simulink model "ABS_VehicleSpeed_Model"  (R2025a)
settings: Solver=VariableStepAuto  StartTime=0.0  StopTime=10.0  RelTol=1e-3
settings Model: Creator=nikul  LastModifiedBy=nikul

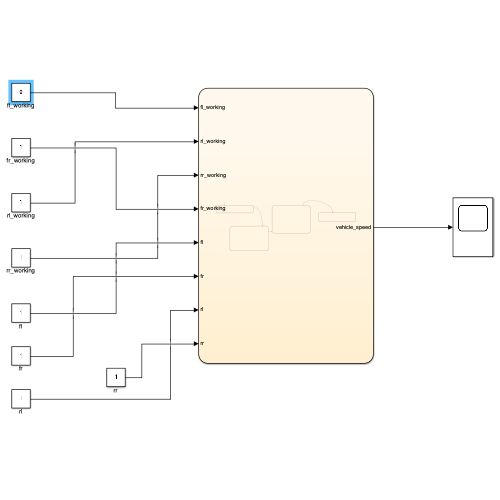
[thumbnail: Simulink's stored preview of the top-level diagram]
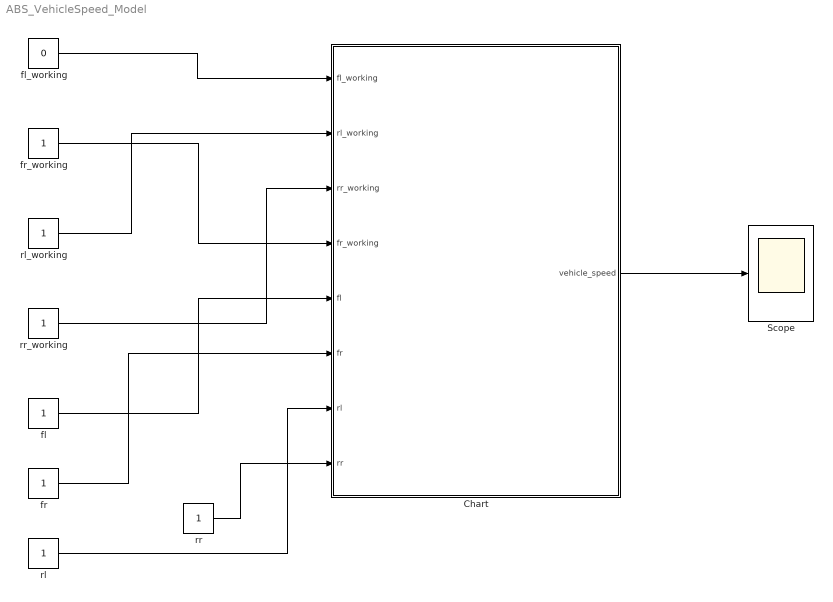
== system ABS_VehicleSpeed_Model ==
  Chart : Stateflow chart  TreatAsAtomicUnit=on
  Scope : Scope
  fl : Constant  OutDataTypeStr=double
  fl_working : Constant  Value=0  OutDataTypeStr=boolean
  fr : Constant  OutDataTypeStr=double
  fr_working : Constant  OutDataTypeStr=boolean
  rl : Constant  OutDataTypeStr=double
  rl_working : Constant  OutDataTypeStr=boolean
  rr : Constant  OutDataTypeStr=double
  rr_working : Constant  OutDataTypeStr=boolean
  wires:
  fl_working/1 -> Chart/1(fl_working)
  fr_working/1 -> Chart/4(fr_working)
  rl_working/1 -> Chart/2(rl_working)
  rr_working/1 -> Chart/3(rr_working)
  fl/1 -> Chart/5(fl)
  fr/1 -> Chart/6(fr)
  rl/1 -> Chart/7(rl)
  rr/1 -> Chart/8(rr)
  Chart/1(vehicle_speed) -> Scope/1

== stateflow chart ABS_VehicleSpeed_Model/Chart ==
  state AllSensorsWorking
    fl_working && fr_working && rl_working && rr_working
    vehicle_speed = (fl + fr + rl + rr) / 4;
  state TwoSensorsDown
    (fl_working + fr_working + rl_working + rr_working) == 2
    if fl_working && fr_working
    vehicle_speed = (fl + fr)/2;
    elseif fl_working && rl_working
    vehicle_speed = (fl + rl)/2;
    elseif fl_working && rr_working
    vehicle_speed = (fl + rr)/2;
    elseif fr_working && rl_working
    vehicle_speed = (fr + rl)/2;
    elseif fr_working && rr_working
    vehicle_speed = (fr + rr)/2;
    elseif rl_working && rr_working
    vehicle_speed = (rl + rr)/2;
    end
  state ThreeOrMoreDown
    (fl_working + fr_working + rl_working + rr_working) <= 1
    vehicle_speed = 0;
  state OneSensorDown
    (~fl_working && fr_working && rl_working && rr_working)
    (~fr_working && fl_working && rl_working && rr_working)
    (~rl_working && fl_working && fr_working && rr_working)
    (~rr_working && fl_working && fr_working && rl_working)
    if ~fl_working
    vehicle_speed = (fr + rl + rr)/3;
    elseif ~fr_working
    vehicle_speed = (fl + rl + rr)/3;
    elseif ~rl_working
    vehicle_speed = (fl + fr + rr)/3;
    elseif ~rr_working
    vehicle_speed = (fl + fr + rl)/3;
    end
  TwoSensorsDown -> ThreeOrMoreDown
  (default) -> AllSensorsWorking
  AllSensorsWorking -> OneSensorDown
  OneSensorDown -> TwoSensorsDown
  data: fl_working input boolean; rl_working input boolean; rr_working input boolean; fr_working input boolean; fl input double; fr input; rl input double; rr input double; vehicle_speed output double
